simulink model "predictor_smith"  (R2024b)
settings: Solver=VariableStepAuto  StartTime=0.0  StopTime=30  RelTol=1e-3
values from neighbouring files (symbols this model uses):
  Kp = Ti/(K_med*Timp)    (= 0.397746967071)    [Fusion_Filtering_TF.m]
  N_dead = round(tau_med/Ts)    [Fusion_Filtering_TF.m]
  tau_med = (tau1 + tau2) / 2    (= 1.65)    [Fusion_Filtering_TF.m]
  Ti = T_med    (= 1.35)    [Fusion_Filtering_TF.m]
libraries: cstblocks x5
settings Model: Creator=justi  LastModifiedBy=justi

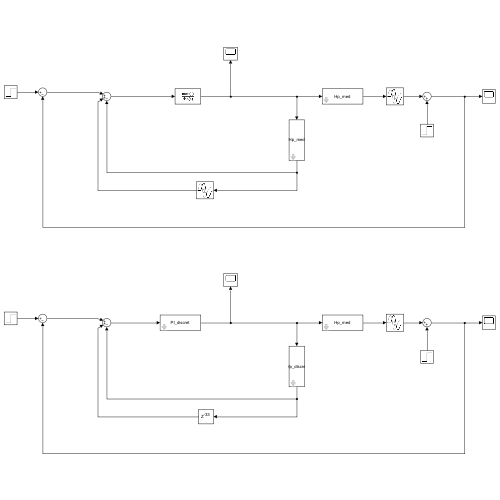
[thumbnail: Simulink's stored preview of the top-level diagram]
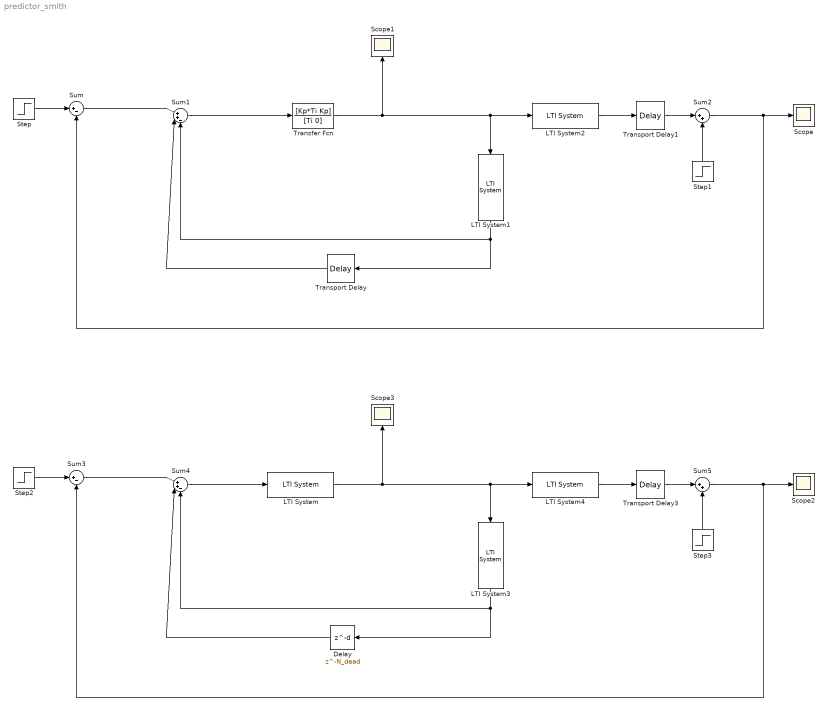
== system predictor_smith ==
  Delay : Delay  DelayLength=N_dead
  LTI System : cstblocks/LTI System  sys=PI_discret  IC=[]  PadeOrder=0
  LTI System1 : cstblocks/LTI System  sys=Hp_med  IC=[]  PadeOrder=0
  LTI System2 : cstblocks/LTI System  sys=Hp_med  IC=[]  PadeOrder=0
  LTI System3 : cstblocks/LTI System  sys=Hp_discret  IC=[]  PadeOrder=0
  LTI System4 : cstblocks/LTI System  sys=Hp_med  IC=[]  PadeOrder=0
  Scope{,1..3} (4 alike) : Scope
  Step : Step  Time=0  After=145  SampleTime=0
  Step1 : Step  Time=20  After=8  SampleTime=0
  Step2 : Step  Time=0  After=145  SampleTime=0
  Step3 : Step  Time=20  After=8  SampleTime=0
  Sum : Sum  Inputs=|+-
  Sum1 : Sum  Inputs=|++-
  Sum2 : Sum  Inputs=|++
  Sum3 : Sum  Inputs=|+-
  Sum4 : Sum  Inputs=|++-
  Sum5 : Sum  Inputs=|++
  Transfer Fcn : TransferFcn  Numerator=[Kp*Ti Kp]  Denominator=[Ti 0]
  Transport Delay : TransportDelay  DelayTime=tau_med
  Transport Delay1 : TransportDelay  DelayTime=tau_med
  Transport Delay3 : TransportDelay  DelayTime=tau_med
  wires:
  Step/1 -> Sum/1
  LTI System2/1 -> Transport Delay1/1
  Transport Delay1/1 -> Sum2/1
  Transfer Fcn/1 -> LTI System1/1, LTI System2/1, Scope1/1
  LTI System1/1 -> Sum1/3, Transport Delay/1
  Transport Delay/1 -> Sum1/2
  Sum/1 -> Sum1/1
  Sum1/1 -> Transfer Fcn/1
  Step1/1 -> Sum2/2
  Sum2/1 -> Sum/2, Scope/1
  LTI System/1 -> LTI System3/1, LTI System4/1, Scope3/1
  Step3/1 -> Sum5/2
  Sum4/1 -> LTI System/1
  Step2/1 -> Sum3/1
  Transport Delay3/1 -> Sum5/1
  LTI System3/1 -> Delay/1, Sum4/3
  Sum3/1 -> Sum4/1
  Delay/1 -> Sum4/2
  LTI System4/1 -> Transport Delay3/1
  Sum5/1 -> Sum3/2, Scope2/1
